simulink model "s_b4a4x64f"  (R2016b)
settings: Solver=VariableStepDiscrete  StartTime=0.0  StopTime=1  RelTol=1e-3
undefined symbols (not defined in the file): fft_stages, n_bits_ants, n_bits_xengs
libraries: xbsIndex_r4 x19869, casper_library_misc x167, casper_library_scopes x10, xbsReplacements_r4 x9, casper_library_delays x8, xps_library x3
(part 12 of 173)

== system s_b4a4x64f/sys3 ==
  note: The time out of the pre_process increments
      | by ONE per freq per fengine.
  31->32 : Subsystem  AncestorBlock=casper_library_bus/bus_convert  mask(bus_convert){n_bits_in=[31 31 31 31 31 31 31 31], bin_pt_in=0, cmplx=off, n_bits_out=32, bin_pt_out=0, quantization=0, overflow=0, latency=0, of=off, misc=off}
      mask prompts: n_bits_in "input bit widths"; bin_pt_in "input binary points"; cmplx "input complex"; n_bits_out "output bit widths"; bin_pt_out "output binary points"; quantization "quantization strategy (Truncate=0, Round  (unbiased: +/- Inf)=1, Round (unbiased: Even Values)=2)"; overflow "overflow strategy (Wrap=0, Saturate=1, Flag as error=2)"; of "overflow indication"; misc "misc support"
      mask help: Convert components of busses
      mask init: same as s_b4a4x64f/sys0/31->32
  Concat1 : xbsIndex_r4/Concat  num_inputs=2  dbl_ovrd=off  block_type=concat
      settings: block_version=10.1.3
  Concat10 : xbsIndex_r4/Concat  num_inputs=2  dbl_ovrd=off  block_type=concat
  Concat11 : xbsIndex_r4/Concat  num_inputs=3  dbl_ovrd=off  block_type=concat
  Concat6 : xbsIndex_r4/Concat  num_inputs=2  dbl_ovrd=off  block_type=concat
  Constant10 : xbsIndex_r4/Constant  const=xeng_id  gui_display_data_type=Fixed-point  arith_type=Unsigned  n_bits=n_bits_xengs_per_fpga  bin_pt=0  preci_type=Single  exp_width=8  frac_width=24  explicit_period=on  period=1  equ=P=C  opselect=C  inp2=PCIN>>17  opr=+  inp1=P  carry=CIN  dbl_ovrd=off  block_type=constant
  Constant11 : xbsIndex_r4/Constant  const=0  gui_display_data_type=Fixed-point  arith_type=Boolean  n_bits=1  bin_pt=0  preci_type=Single  exp_width=8  frac_width=24  explicit_period=on  period=1  equ=P=C  opselect=C  inp2=PCIN>>17  opr=+  inp1=P  carry=CIN  dbl_ovrd=off  block_type=constant
      settings: block_version=11.3
  Constant12 : xbsIndex_r4/Constant  const=0  gui_display_data_type=Fixed-point  arith_type=Boolean  n_bits=1  bin_pt=0  preci_type=Single  exp_width=8  frac_width=24  explicit_period=on  period=1  equ=P=C  opselect=C  inp2=PCIN>>17  opr=+  inp1=P  carry=CIN  dbl_ovrd=off  block_type=constant
      settings: block_version=11.3
  Constant13 : xbsIndex_r4/Constant  const=0  gui_display_data_type=Fixed-point  arith_type=Unsigned  n_bits=n_bits_channels + 1 + x_acc_bits  bin_pt=0  preci_type=Single  exp_width=8  frac_width=24  explicit_period=on  period=1  equ=P=C  opselect=C  inp2=PCIN>>17  opr=+  inp1=P  carry=CIN  dbl_ovrd=off  block_type=constant
  Constant14 : xbsIndex_r4/Constant  const=0  gui_display_data_type=Fixed-point  arith_type=Unsigned  n_bits=16  bin_pt=0  preci_type=Single  exp_width=8  frac_width=24  explicit_period=on  period=1  equ=P=C  opselect=C  inp2=PCIN>>17  opr=+  inp1=P  carry=CIN  dbl_ovrd=off  block_type=constant
  Constant15 : xbsIndex_r4/Constant  const=0  gui_display_data_type=Fixed-point  arith_type=Unsigned  n_bits=16-n_bits_channels  bin_pt=0  preci_type=Single  exp_width=8  frac_width=24  explicit_period=on  period=1  equ=P=C  opselect=C  inp2=PCIN>>17  opr=+  inp1=P  carry=CIN  dbl_ovrd=off  block_type=constant
  Constant5 : xbsIndex_r4/Constant  const=0  gui_display_data_type=Fixed-point  arith_type=Unsigned  n_bits=n_bits_channels + 1 + x_acc_bits  bin_pt=0  preci_type=Single  exp_width=8  frac_width=24  explicit_period=on  period=1  equ=P=C  opselect=C  inp2=PCIN>>17  opr=+  inp1=P  carry=CIN  dbl_ovrd=off  block_type=constant
  Delay{1..4} (4 alike) : xbsIndex_r4/Delay  rst=off  infoeditControl=Selection of Reset will increase slice count due to use of real FFs and instead of SRLs  en=on  latency=1  reg_retiming=on  dbl_ovrd=off  block_type=delay
  Delay10 : Subsystem  AncestorBlock=casper_library_delays/pipeline  mask(pipeline){latency=2}
      mask help:
      | An explicitly laid-out delay line to avoid mapping to SRL16s
      | for use in pipelining to help achieve timing closure.
      mask init:
      | pipeline_init(gcb,'latency',latency);
      settings: AttributesFormatString=Latency = %<latency>
      mask Display:
      | port_label('input', 1, 'd');
      | port_label('output', 1, 'q');
      | disp(['Z^-', num2str(latency)]);
  Delay11 : Subsystem  AncestorBlock=casper_library_delays/pipeline  mask(pipeline){latency=2}
      mask help:
      | An explicitly laid-out delay line to avoid mapping to SRL16s
      | for use in pipelining to help achieve timing closure.
      mask init:
      | pipeline_init(gcb,'latency',latency);
      settings: AttributesFormatString=Latency = %<latency>
      mask Display:
      | port_label('input', 1, 'd');
      | port_label('output', 1, 'q');
      | disp(['Z^-', num2str(latency)]);
  Delay12 : Subsystem  AncestorBlock=casper_library_delays/pipeline  mask(pipeline){latency=2}
      mask help:
      | An explicitly laid-out delay line to avoid mapping to SRL16s
      | for use in pipelining to help achieve timing closure.
      mask init:
      | pipeline_init(gcb,'latency',latency);
      settings: AttributesFormatString=Latency = %<latency>
      mask Display:
      | port_label('input', 1, 'd');
      | port_label('output', 1, 'q');
      | disp(['Z^-', num2str(latency)]);
  Delay13 : Subsystem  AncestorBlock=casper_library_delays/pipeline  mask(pipeline){latency=2}
      mask help:
      | An explicitly laid-out delay line to avoid mapping to SRL16s
      | for use in pipelining to help achieve timing closure.
      mask init:
      | pipeline_init(gcb,'latency',latency);
      settings: AttributesFormatString=Latency = %<latency>
      mask Display:
      | port_label('input', 1, 'd');
      | port_label('output', 1, 'q');
      | disp(['Z^-', num2str(latency)]);
  Delay14 : Subsystem  AncestorBlock=casper_library_delays/pipeline  mask(pipeline){latency=2}
      mask help:
      | An explicitly laid-out delay line to avoid mapping to SRL16s
      | for use in pipelining to help achieve timing closure.
      mask init:
      | pipeline_init(gcb,'latency',latency);
      settings: AttributesFormatString=Latency = %<latency>
      mask Display:
      | port_label('input', 1, 'd');
      | port_label('output', 1, 'q');
      | disp(['Z^-', num2str(latency)]);
  Delay15 : Subsystem  AncestorBlock=casper_library_delays/pipeline  mask(pipeline){latency=2}
      mask help:
      | An explicitly laid-out delay line to avoid mapping to SRL16s
      | for use in pipelining to help achieve timing closure.
      mask init:
      | pipeline_init(gcb,'latency',latency);
      settings: AttributesFormatString=Latency = %<latency>
      mask Display:
      | port_label('input', 1, 'd');
      | port_label('output', 1, 'q');
      | disp(['Z^-', num2str(latency)]);
  Delay16 : Subsystem  AncestorBlock=casper_library_delays/pipeline  mask(pipeline){latency=2}
      mask help:
      | An explicitly laid-out delay line to avoid mapping to SRL16s
      | for use in pipelining to help achieve timing closure.
      mask init:
      | pipeline_init(gcb,'latency',latency);
      settings: AttributesFormatString=Latency = %<latency>
      mask Display:
      | port_label('input', 1, 'd');
      | port_label('output', 1, 'q');
      | disp(['Z^-', num2str(latency)]);
  Delay17 : Subsystem  AncestorBlock=casper_library_delays/pipeline  mask(pipeline){latency=2}
      mask help:
      | An explicitly laid-out delay line to avoid mapping to SRL16s
      | for use in pipelining to help achieve timing closure.
      mask init:
      | pipeline_init(gcb,'latency',latency);
      settings: AttributesFormatString=Latency = %<latency>
      mask Display:
      | port_label('input', 1, 'd');
      | port_label('output', 1, 'q');
      | disp(['Z^-', num2str(latency)]);
  Delay18 : Subsystem  AncestorBlock=casper_library_delays/pipeline  mask(pipeline){latency=2}
      mask help:
      | An explicitly laid-out delay line to avoid mapping to SRL16s
      | for use in pipelining to help achieve timing closure.
      mask init:
      | pipeline_init(gcb,'latency',latency);
      settings: AttributesFormatString=Latency = %<latency>
      mask Display:
      | port_label('input', 1, 'd');
      | port_label('output', 1, 'q');
      | disp(['Z^-', num2str(latency)]);
  Delay19 : Subsystem  AncestorBlock=casper_library_delays/pipeline  mask(pipeline){latency=2}
      mask help:
      | An explicitly laid-out delay line to avoid mapping to SRL16s
      | for use in pipelining to help achieve timing closure.
      mask init:
      | pipeline_init(gcb,'latency',latency);
      settings: AttributesFormatString=Latency = %<latency>
      mask Display:
      | port_label('input', 1, 'd');
      | port_label('output', 1, 'q');
      | disp(['Z^-', num2str(latency)]);
  Delay20 : Subsystem  AncestorBlock=casper_library_delays/pipeline  mask(pipeline){latency=2}
      mask help:
      | An explicitly laid-out delay line to avoid mapping to SRL16s
      | for use in pipelining to help achieve timing closure.
      mask init:
      | pipeline_init(gcb,'latency',latency);
      settings: AttributesFormatString=Latency = %<latency>
      mask Display:
      | port_label('input', 1, 'd');
      | port_label('output', 1, 'q');
      | disp(['Z^-', num2str(latency)]);
  Delay21 : Subsystem  AncestorBlock=casper_library_delays/pipeline  mask(pipeline){latency=2}
      mask help:
      | An explicitly laid-out delay line to avoid mapping to SRL16s
      | for use in pipelining to help achieve timing closure.
      mask init:
      | pipeline_init(gcb,'latency',latency);
      settings: AttributesFormatString=Latency = %<latency>
      mask Display:
      | port_label('input', 1, 'd');
      | port_label('output', 1, 'q');
      | disp(['Z^-', num2str(latency)]);
  Delay22 : Subsystem  AncestorBlock=casper_library_delays/pipeline  mask(pipeline){latency=2}
      mask help:
      | An explicitly laid-out delay line to avoid mapping to SRL16s
      | for use in pipelining to help achieve timing closure.
      mask init:
      | pipeline_init(gcb,'latency',latency);
      settings: AttributesFormatString=Latency = %<latency>
      mask Display:
      | port_label('input', 1, 'd');
      | port_label('output', 1, 'q');
      | disp(['Z^-', num2str(latency)]);
  Delay23 : Subsystem  AncestorBlock=casper_library_delays/pipeline  mask(pipeline){latency=2}
      mask help:
      | An explicitly laid-out delay line to avoid mapping to SRL16s
      | for use in pipelining to help achieve timing closure.
      mask init:
      | pipeline_init(gcb,'latency',latency);
      settings: AttributesFormatString=Latency = %<latency>
      mask Display:
      | port_label('input', 1, 'd');
      | port_label('output', 1, 'q');
      | disp(['Z^-', num2str(latency)]);
  Delay{6..7,32..34,68,71,93} (8 alike) : xbsIndex_r4/Delay  rst=off  infoeditControl=Selection of Reset will increase slice count due to use of real FFs and instead of SRLs  en=off  latency=1  reg_retiming=on  dbl_ovrd=off  block_type=delay
      Delay32 settings: block_version=11.4
      Delay33 settings: block_version=11.4
      Delay34 settings: block_version=11.4
      Delay68 settings: block_version=11.4
      Delay71 settings: block_version=11.4
      Delay93 settings: block_version=11.4
  Delay37 : Subsystem  AncestorBlock=casper_library_delays/pipeline  mask(pipeline){latency=1}
      mask help:
      | An explicitly laid-out delay line to avoid mapping to SRL16s
      | for use in pipelining to help achieve timing closure.
      mask init:
      | pipeline_init(gcb,'latency',latency);
      settings: AttributesFormatString=Latency = %<latency>
      mask Display:
      | port_label('input', 1, 'd');
      | port_label('output', 1, 'q');
      | disp(['Z^-', num2str(latency)]);
  Delay38 : Subsystem  AncestorBlock=casper_library_delays/pipeline  mask(pipeline){latency=1}
      mask help:
      | An explicitly laid-out delay line to avoid mapping to SRL16s
      | for use in pipelining to help achieve timing closure.
      mask init:
      | pipeline_init(gcb,'latency',latency);
      settings: AttributesFormatString=Latency = %<latency>
      mask Display:
      | port_label('input', 1, 'd');
      | port_label('output', 1, 'q');
      | disp(['Z^-', num2str(latency)]);
  Delay{5,81,90..91} (4 alike) : xbsIndex_r4/Delay  rst=off  infoeditControl=Selection of Reset will increase slice count due to use of real FFs and instead of SRLs  en=off  latency=2  reg_retiming=off  dbl_ovrd=off  block_type=delay
      settings: infoedit=Hardware notes: A delay line is a chain, each link of which is an SRL16 or SRL32 followed by a flip-flop.  xl_area=[0, 0, 0, 0, 0, 0, 0]  block_version=9.2.01
  Delay52 : Subsystem  AncestorBlock=casper_library_delays/pipeline  mask(pipeline){latency=1}
      mask help:
      | An explicitly laid-out delay line to avoid mapping to SRL16s
      | for use in pipelining to help achieve timing closure.
      mask init:
      | pipeline_init(gcb,'latency',latency);
      settings: AttributesFormatString=Latency = %<latency>
      mask Display:
      | port_label('input', 1, 'd');
      | port_label('output', 1, 'q');
      | disp(['Z^-', num2str(latency)]);
  Delay69 : Subsystem  AncestorBlock=casper_library_delays/pipeline  mask(pipeline){latency=2}
      mask help:
      | An explicitly laid-out delay line to avoid mapping to SRL16s
      | for use in pipelining to help achieve timing closure.
      mask init:
      | pipeline_init(gcb,'latency',latency);
      settings: AttributesFormatString=Latency = %<latency>
      mask Display:
      | port_label('input', 1, 'd');
      | port_label('output', 1, 'q');
      | disp(['Z^-', num2str(latency)]);
  Delay74 : Subsystem  AncestorBlock=casper_library_delays/pipeline  mask(pipeline){latency=2}
      mask help:
      | An explicitly laid-out delay line to avoid mapping to SRL16s
      | for use in pipelining to help achieve timing closure.
      mask init:
      | pipeline_init(gcb,'latency',latency);
      settings: AttributesFormatString=Latency = %<latency>
      mask Display:
      | port_label('input', 1, 'd');
      | port_label('output', 1, 'q');
      | disp(['Z^-', num2str(latency)]);
  Delay76 : Subsystem  AncestorBlock=casper_library_delays/pipeline  mask(pipeline){latency=2}
      mask help:
      | An explicitly laid-out delay line to avoid mapping to SRL16s
      | for use in pipelining to help achieve timing closure.
      mask init:
      | pipeline_init(gcb,'latency',latency);
      settings: AttributesFormatString=Latency = %<latency>
      mask Display:
      | port_label('input', 1, 'd');
      | port_label('output', 1, 'q');
      | disp(['Z^-', num2str(latency)]);
  Delay77 : Subsystem  AncestorBlock=casper_library_delays/pipeline  mask(pipeline){latency=2}
      mask help:
      | An explicitly laid-out delay line to avoid mapping to SRL16s
      | for use in pipelining to help achieve timing closure.
      mask init:
      | pipeline_init(gcb,'latency',latency);
      settings: AttributesFormatString=Latency = %<latency>
      mask Display:
      | port_label('input', 1, 'd');
      | port_label('output', 1, 'q');
      | disp(['Z^-', num2str(latency)]);
  Delay8 : Subsystem  AncestorBlock=casper_library_delays/pipeline  mask(pipeline){latency=1}
      mask help:
      | An explicitly laid-out delay line to avoid mapping to SRL16s
      | for use in pipelining to help achieve timing closure.
      mask init:
      | pipeline_init(gcb,'latency',latency);
      settings: AttributesFormatString=Latency = %<latency>
      mask Display:
      | port_label('input', 1, 'd');
      | port_label('output', 1, 'q');
      | disp(['Z^-', num2str(latency)]);
  Delay89 : Subsystem  AncestorBlock=casper_library_delays/pipeline  mask(pipeline){latency=2}
      mask help:
      | An explicitly laid-out delay line to avoid mapping to SRL16s
      | for use in pipelining to help achieve timing closure.
      mask init:
      | pipeline_init(gcb,'latency',latency);
      settings: AttributesFormatString=Latency = %<latency>
      mask Display:
      | port_label('input', 1, 'd');
      | port_label('output', 1, 'q');
      | disp(['Z^-', num2str(latency)]);
  Delay9 : Subsystem  AncestorBlock=casper_library_delays/pipeline  mask(pipeline){latency=2}
      mask help:
      | An explicitly laid-out delay line to avoid mapping to SRL16s
      | for use in pipelining to help achieve timing closure.
      mask init:
      | pipeline_init(gcb,'latency',latency);
      settings: AttributesFormatString=Latency = %<latency>
      mask Display:
      | port_label('input', 1, 'd');
      | port_label('output', 1, 'q');
      | disp(['Z^-', num2str(latency)]);
  Inverter : xbsIndex_r4/Inverter  en=off  latency=0  dbl_ovrd=off  block_type=inv
  Inverter2 : xbsIndex_r4/Inverter  en=off  latency=0  dbl_ovrd=off  block_type=inv
  Inverter3 : xbsIndex_r4/Inverter  en=off  latency=0  dbl_ovrd=off  block_type=inv
  Logical : xbsIndex_r4/Logical  logical_function=AND  inputs=2  en=off  latency=0  precision=Full  arith_type=Unsigned  n_bits=16  bin_pt=0  align_bp=on  dbl_ovrd=off  block_type=logical
  Logical1 : xbsIndex_r4/Logical  logical_function=AND  inputs=2  en=off  latency=1  precision=Full  arith_type=Unsigned  n_bits=16  bin_pt=0  align_bp=on  dbl_ovrd=off  block_type=logical
  Mux : xbsIndex_r4/Mux  inputs=2  en=off  latency=1  precision=Full  arith_type=Unsigned  n_bits=16  bin_pt=14  quantization=Truncate  overflow=Wrap  dbl_ovrd=off  block_type=mux
  Register : xbsIndex_r4/Register  init=0  rst=off  en=on  dbl_ovrd=off  block_type=register
  Register2 : xbsIndex_r4/Register  init=0  rst=off  en=on  dbl_ovrd=off  block_type=register
      settings: block_version=11.4
  Register3 : xbsIndex_r4/Register  init=0  rst=off  en=on  dbl_ovrd=off  block_type=register
      settings: block_version=11.4
  Slice1 : xbsIndex_r4/Slice  nbits=timestamp_bits  boolean_output=off  mode=Upper Bit Location + Width  bit1=0  base1=MSB of Input  bit0=timestamp_bits  base0=LSB of Input  dbl_ovrd=off  block_type=slice
  Slice11 : xbsIndex_r4/Slice  nbits=n_bits_xengs - n_bits_xengs_per_fpga  boolean_output=off  mode=Lower Bit Location + Width  bit1=0  base1=MSB of Input  bit0=0  base0=LSB of Input  dbl_ovrd=off  block_type=slice
      settings: block_version=10.1.3
  Slice12 : xbsIndex_r4/Slice  nbits=16  boolean_output=off  mode=Lower Bit Location + Width  bit1=0  base1=MSB of Input  bit0=0  base0=LSB of Input  dbl_ovrd=off  block_type=slice
  Slice15 : xbsIndex_r4/Slice  nbits=1  boolean_output=on  mode=Upper Bit Location + Width  bit1=0  base1=MSB of Input  bit0=0  base0=LSB of Input  dbl_ovrd=off  block_type=slice
  Slice16 : xbsIndex_r4/Slice  nbits=1  boolean_output=on  mode=Lower Bit Location + Width  bit1=0  base1=LSB of Input  bit0=0  base0=LSB of Input  dbl_ovrd=off  block_type=slice
  Slice2 : xbsIndex_r4/Slice  nbits=16  boolean_output=off  mode=Upper Bit Location + Width  bit1=0  base1=MSB of Input  bit0=0  base0=LSB of Input  dbl_ovrd=off  block_type=slice
  Terminator2 : Terminator
  bf : Subsystem  mask{beng_bits=n_bits_xengs, ant_bits=n_bits_ants, polarisation_bits=1, freq_bits=n_bits_channels, stack_bits=x_acc_bits, n_bits_in=8, bin_pt_in=7, bfpga_bits=2, timestamp_bits=timestamp_bits, n_bits_norm=16, bin_pt_norm=9, n_bits_combine=8+16+1+n_bits_ants, n_bits_requant=16, bin_pt_requant=8, bram_latency=5, add_latency=3, mult_latency=5, beam_bits=0, n_bits_out=8, bin_pt_out=7, conv_latency=3, output_enabled=on}
      mask prompts: beng_bits "b-engines (2^?)"; ant_bits "antennas (2^?)"; polarisation_bits "polarisations (2^?)"; freq_bits "frequencies (2^?)"; stack_bits "stacking factor (2^?)"; n_bits_in "data bits in"; bin_pt_in "binary point in"; bfpga_bits "b-engines on FPGA"; timestamp_bits "timestamp size (bits)"; n_bits_norm "calibration factor data bits"; bin_pt_norm "calibration factor binary point"; n_bits_combine "antenna combination output bit width"; n_bits_requant "requantization factor bit width"; bin_pt_requant "requantization factor binary point"; bram_latency "bram latency"; add_latency "add latency"; beam_bits "beams (2^?)"; n_bits_out "data bits out"; bin_pt_out "binary point out"; conv_latency "convert latency"; output_enabled "output enabled by default?"
      mask help:
      | Frequency domain beamformer
      |
      | b-engines: number of b-engines in system (same as x-engines)
      | stacking factor: the number of consecutive time samples in a data block
      | calibration factor: the complex factor multiplied with the incoming data.
      | The complex value is unique to each beam, input and frequency.
      | Requantization factor: real factor multiplied with the output data before
      | quantization. The value is unique to each beam and frequency.
      | beams: the number of beams per polarisation
      | ouput enabled by default: can be useful for simulation
      mask init:
      | set_param([gcb,'/fbf'], ...
      |     'output_enabled', output_enabled);
      mask Help:
      | Accepts the same channelised data as the CASPER FX correlator x-engine core.
      | Polarisations appear in order in different beams. (for polarisation (0,1), 0 in [0,2...], 1 in [1,3...]).
      | TODO: beam steering.
      | TODO: Stokes output.
      | TODO: accumulation.
  bf_pack_out0 : Subsystem  mask(speadify){spead_msw=64, spead_lsw=48, heap_bits=n_bits_channels-n_bits_xengs+x_acc_bits, group_size_bits=n_bits_xengs, n_bits_chans=n_bits_channels-n_bits_xengs, n_bits_acc=x_acc_bits, bit_width_in=1, bit_width_out=5, packet_bits=12, fabric_clock=225, tx_clock=156.25}
      mask prompts: spead_msw "SPEAD flavour (msw)"; spead_lsw "SPEAD flavour (lsw)"; heap_bits "heap size (2^? input words)"; group_size_bits "max SPEAD heap group size (2^?)"; n_bits_chans "channels processed (2^?)"; n_bits_acc "samples from channel (2^?)"; bit_width_in "word size in (2^? bytes)"; bit_width_out "word size out (2^? bytes)"; packet_bits "packet size out (2^? bytes)"; fabric_clock "fabric clock (MHz)"; tx_clock "transmission clock (MHz)"
      mask help:
      | Transforms input data stream to 10Ge ready SPEAD stream.
      | max SPEAD heap group size is the maximum number of SPEAD sources
      | that may be combined when assembling heaps. n_partitions and partition
      | input ports are then used at runtime to configure this.
  bf_pack_out1 : Subsystem  mask(speadify){spead_msw=64, spead_lsw=48, heap_bits=n_bits_channels-n_bits_xengs+x_acc_bits, group_size_bits=n_bits_xengs, n_bits_chans=n_bits_channels-n_bits_xengs, n_bits_acc=x_acc_bits, bit_width_in=1, bit_width_out=5, packet_bits=12, fabric_clock=225, tx_clock=156.25}
      mask prompts: spead_msw "SPEAD flavour (msw)"; spead_lsw "SPEAD flavour (lsw)"; heap_bits "heap size (2^? input words)"; group_size_bits "max SPEAD heap group size (2^?)"; n_bits_chans "channels processed (2^?)"; n_bits_acc "samples from channel (2^?)"; bit_width_in "word size in (2^? bytes)"; bit_width_out "word size out (2^? bytes)"; packet_bits "packet size out (2^? bytes)"; fabric_clock "fabric clock (MHz)"; tx_clock "transmission clock (MHz)"
      mask help:
      | Transforms input data stream to 10Ge ready SPEAD stream.
      | max SPEAD heap group size is the maximum number of SPEAD sources
      | that may be combined when assembling heaps. n_partitions and partition
      | input ports are then used at runtime to configure this.
  pipeline : Subsystem  AncestorBlock=casper_library_delays/pipeline  mask(pipeline){latency=2}
      mask help:
      | An explicitly laid-out delay line to avoid mapping to SRL16s
      | for use in pipelining to help achieve timing closure.
      mask init:
      | pipeline_init(gcb,'latency',latency);
      settings: AttributesFormatString=Latency = %<latency>
      mask Display:
      | port_label('input', 1, 'd');
      | port_label('output', 1, 'q');
      | disp(['Z^-', num2str(latency)]);
  pipeline1 : Subsystem  AncestorBlock=casper_library_delays/pipeline  mask(pipeline){latency=2}
      mask help:
      | An explicitly laid-out delay line to avoid mapping to SRL16s
      | for use in pipelining to help achieve timing closure.
      mask init:
      | pipeline_init(gcb,'latency',latency);
      settings: AttributesFormatString=Latency = %<latency>
      mask Display:
      | port_label('input', 1, 'd');
      | port_label('output', 1, 'q');
      | disp(['Z^-', num2str(latency)]);
  pipeline10 : Subsystem  AncestorBlock=casper_library_delays/pipeline  mask(pipeline){latency=2}
      mask help:
      | An explicitly laid-out delay line to avoid mapping to SRL16s
      | for use in pipelining to help achieve timing closure.
      mask init:
      | pipeline_init(gcb,'latency',latency);
      settings: AttributesFormatString=Latency = %<latency>
      mask Display:
      | port_label('input', 1, 'd');
      | port_label('output', 1, 'q');
      | disp(['Z^-', num2str(latency)]);
  pipeline11 : Subsystem  AncestorBlock=casper_library_delays/pipeline  mask(pipeline){latency=2}
      mask help:
      | An explicitly laid-out delay line to avoid mapping to SRL16s
      | for use in pipelining to help achieve timing closure.
      mask init:
      | pipeline_init(gcb,'latency',latency);
      settings: AttributesFormatString=Latency = %<latency>
      mask Display:
      | port_label('input', 1, 'd');
      | port_label('output', 1, 'q');
      | disp(['Z^-', num2str(latency)]);
  pipeline12 : Subsystem  AncestorBlock=casper_library_delays/pipeline  mask(pipeline){latency=2}
      mask help:
      | An explicitly laid-out delay line to avoid mapping to SRL16s
      | for use in pipelining to help achieve timing closure.
      mask init:
      | pipeline_init(gcb,'latency',latency);
      settings: AttributesFormatString=Latency = %<latency>
      mask Display:
      | port_label('input', 1, 'd');
      | port_label('output', 1, 'q');
      | disp(['Z^-', num2str(latency)]);
  pipeline13 : Subsystem  AncestorBlock=casper_library_delays/pipeline  mask(pipeline){latency=2}
      mask help:
      | An explicitly laid-out delay line to avoid mapping to SRL16s
      | for use in pipelining to help achieve timing closure.
      mask init:
      | pipeline_init(gcb,'latency',latency);
      settings: AttributesFormatString=Latency = %<latency>
      mask Display:
      | port_label('input', 1, 'd');
      | port_label('output', 1, 'q');
      | disp(['Z^-', num2str(latency)]);
  pipeline14 : Subsystem  AncestorBlock=casper_library_delays/pipeline  mask(pipeline){latency=2}
      mask help:
      | An explicitly laid-out delay line to avoid mapping to SRL16s
      | for use in pipelining to help achieve timing closure.
      mask init:
      | pipeline_init(gcb,'latency',latency);
      settings: AttributesFormatString=Latency = %<latency>
      mask Display:
      | port_label('input', 1, 'd');
      | port_label('output', 1, 'q');
      | disp(['Z^-', num2str(latency)]);
  pipeline2 : Subsystem  AncestorBlock=casper_library_delays/pipeline  mask(pipeline){latency=2}
      mask help:
      | An explicitly laid-out delay line to avoid mapping to SRL16s
      | for use in pipelining to help achieve timing closure.
      mask init:
      | pipeline_init(gcb,'latency',latency);
      settings: AttributesFormatString=Latency = %<latency>
      mask Display:
      | port_label('input', 1, 'd');
      | port_label('output', 1, 'q');
      | disp(['Z^-', num2str(latency)]);
  pipeline3 : Subsystem  AncestorBlock=casper_library_delays/pipeline  mask(pipeline){latency=2}
      mask help:
      | An explicitly laid-out delay line to avoid mapping to SRL16s
      | for use in pipelining to help achieve timing closure.
      mask init:
      | pipeline_init(gcb,'latency',latency);
      settings: AttributesFormatString=Latency = %<latency>
      mask Display:
      | port_label('input', 1, 'd');
      | port_label('output', 1, 'q');
      | disp(['Z^-', num2str(latency)]);
  pipeline4 : Subsystem  AncestorBlock=casper_library_delays/pipeline  mask(pipeline){latency=2}
      mask help:
      | An explicitly laid-out delay line to avoid mapping to SRL16s
      | for use in pipelining to help achieve timing closure.
      mask init:
      | pipeline_init(gcb,'latency',latency);
      settings: AttributesFormatString=Latency = %<latency>
      mask Display:
      | port_label('input', 1, 'd');
      | port_label('output', 1, 'q');
      | disp(['Z^-', num2str(latency)]);
  pipeline5 : Subsystem  AncestorBlock=casper_library_delays/pipeline  mask(pipeline){latency=2}
      mask help:
      | An explicitly laid-out delay line to avoid mapping to SRL16s
      | for use in pipelining to help achieve timing closure.
      mask init:
      | pipeline_init(gcb,'latency',latency);
      settings: AttributesFormatString=Latency = %<latency>
      mask Display:
      | port_label('input', 1, 'd');
      | port_label('output', 1, 'q');
      | disp(['Z^-', num2str(latency)]);
  pipeline6 : Subsystem  AncestorBlock=casper_library_delays/pipeline  mask(pipeline){latency=2}
      mask help:
      | An explicitly laid-out delay line to avoid mapping to SRL16s
      | for use in pipelining to help achieve timing closure.
      mask init:
      | pipeline_init(gcb,'latency',latency);
      settings: AttributesFormatString=Latency = %<latency>
      mask Display:
      | port_label('input', 1, 'd');
      | port_label('output', 1, 'q');
      | disp(['Z^-', num2str(latency)]);
  pipeline7 : Subsystem  AncestorBlock=casper_library_delays/pipeline  mask(pipeline){latency=2}
      mask help:
      | An explicitly laid-out delay line to avoid mapping to SRL16s
      | for use in pipelining to help achieve timing closure.
      mask init:
      | pipeline_init(gcb,'latency',latency);
      settings: AttributesFormatString=Latency = %<latency>
      mask Display:
      | port_label('input', 1, 'd');
      | port_label('output', 1, 'q');
      | disp(['Z^-', num2str(latency)]);
  pipeline8 : Subsystem  AncestorBlock=casper_library_delays/pipeline  mask(pipeline){latency=2}
      mask help:
      | An explicitly laid-out delay line to avoid mapping to SRL16s
      | for use in pipelining to help achieve timing closure.
      mask init:
      | pipeline_init(gcb,'latency',latency);
      settings: AttributesFormatString=Latency = %<latency>
      mask Display:
      | port_label('input', 1, 'd');
      | port_label('output', 1, 'q');
      | disp(['Z^-', num2str(latency)]);
  pipeline9 : Subsystem  AncestorBlock=casper_library_delays/pipeline  mask(pipeline){latency=2}
      mask help:
      | An explicitly laid-out delay line to avoid mapping to SRL16s
      | for use in pipelining to help achieve timing closure.
      mask init:
      | pipeline_init(gcb,'latency',latency);
      settings: AttributesFormatString=Latency = %<latency>
      mask Display:
      | port_label('input', 1, 'd');
      | port_label('output', 1, 'q');
      | disp(['Z^-', num2str(latency)]);
  pkt_reord : Subsystem  mask{ant_bits=n_bits_ants, xeng_bits=n_bits_xengs, chan_bits=n_bits_channels, x_int_bits=x_acc_bits, window_bits=2, min_sync_bits=x_acc_bits+(n_bits_channels-n_bits_xengs)+3, n_bits_timestamp=timestamp_bits, n_bits_data=32, n_bits_input_words=3, n_bits_output_words=0}
      mask prompts: ant_bits "Maximum Number of Antennas (2^?):"; xeng_bits "Number of Xengines in the system (2^?)"; chan_bits "Number of frequency channels in the system (2^?)"; x_int_bits "X Engine Integration Length (2^?):"; window_bits "Number of Windows to Buffer (2^?):"; min_sync_bits "Minimum sync period (2^n)"; n_bits_timestamp "Timestamp bit width"; n_bits_data "Input data word width"; n_bits_input_words "Input data words (2^?)"; n_bits_output_words "Output data words (2^?)"
      mask init: same as s_b4a4x64f/sys0/pkt_reord
      settings: AttributesFormatString=|
      | Sync period: 2^17
      | Payload Len: 64
  pre_process : Subsystem  mask{share_bits=2, xeng_bits=n_bits_xengs, freq_bits=n_bits_channels, acc_bits=x_acc_bits, time_bits=3, ant_bits=n_bits_ants}
      mask prompts: share_bits "Number of X-engines on this link (2^N)?"; xeng_bits "Number of X-engines in system (2^N)?"; freq_bits "Number of frequency channels in system (2^N)?"; acc_bits "xengine accumulation length (2^?)"; time_bits "samples per timestamp increment (2^?)"; ant_bits "max number of antennas in system (2^?)"
  vacc : Subsystem  Tag=casper:vacc  mask{ants_bits=n_bits_ants, freq_bits=fft_stages-1, xeng_bits=n_bits_xengs, acc_bits=x_acc_bits, tick_bits=0, mezz=1, n_inputs=3, n_bits=31, n_bits_flags=ones(1,19)}
      mask prompts: ants_bits "Number of antennas (2^n)"; freq_bits "Number of frequency channels (2^n)"; xeng_bits "Number of X engines (2^n)"; acc_bits "Pre-accumulation in xengine (2^?)"; tick_bits "Timestamp samples per tick (2^?)"; mezz "HMC Mezz site"; n_inputs "Simultaneous inputs (2^?)"; n_bits "Data width (bits)"; n_bits_flags "Flag bit widths"
      mask help: Hardcoded for X engines with a demux of 8!
      mask init: same as s_b4a4x64f/sys0/vacc
      settings: AttributesFormatString=Vector Length: 640
      mask TypeOptions mezz: 0 | 1 | 2 | 3
  vacc_tvg : Subsystem  AncestorBlock=casper_library/Accumulators/vacc_tvg  mask{len=(2^n_bits_ants*(2^n_bits_ants+1))/2*8*2^(n_bits_channels-n_bits_xengs), n_bits=32, n_inputs=8}
      mask prompts: len "Number of Vectors"; n_bits "Data bits"; n_inputs "Simultaneous inputs"
      mask init:
      | fmtstr = sprintf('Vector Length: %d', len/n_inputs);
      | set_param(gcb, 'AttributesFormatString', fmtstr);
      settings: AttributesFormatString=Vector Length: 640
  x_cast : Subsystem  mask{n_bits_in=32, n_bits_out=31, fix_pnt_pos=0, demux_factor=1}
      mask prompts: n_bits_in "Number of bits (input)"; n_bits_out "Number of bits (output)"; fix_pnt_pos "Fixed point position"; demux_factor "Demux Factor"
      mask init: same as s_b4a4x64f/sys0/x_cast
      settings: AttributesFormatString=32 -> 31, demux 1.
  xeng : Subsystem  Tag=casper:xeng  AncestorBlock=casper_library_correlator/xeng  mask(xeng){n_ants=2^n_bits_ants, n_bits=8, acc_len=2^x_acc_bits, demux_factor=1, add_latency=3, mult_latency=4, bram_latency=7, use_ded_mult=1, use_bram_delay=1}
      mask prompts: n_ants "Number of antennas"; n_bits "Bit-width of samples in"; acc_len "Accumulation length"; add_latency "Adder latency"; mult_latency "Multiplier latency"; bram_latency "BRAM latency"; use_ded_mult "Implementation: Multiplier type (0=slices 1=embedded 2=bram)"; use_bram_delay "Implementation: Delay type (0=SLR, 1=BRAM)"
      mask help: CASPER X engine with added internal valid data masking functionality, descramble and integral demux. Based on Aaron Parsons' and Lynn Urry's original X engine design.
      mask init: same as s_b4a4x64f/sys0/xeng
      settings: AttributesFormatString=n_ant=4, bits=8, mult_typ=1, bram_typ=1
      mask TypeOptions demux_factor: 1 | 2 | 4 | 8
  xeng_pack_out : Subsystem  mask(pkt_pack_mask){vector_len=(2^n_bits_ants*(2^n_bits_ants+1))/2*8*2^(n_bits_channels-n_bits_xengs)/8, n_bits_chans=n_bits_channels-n_bits_xengs, n_bits_word_size=5, heap_len=(2^n_bits_ants*(2^n_bits_ants+1))/2*8*(2^(n_bits_channels-n_bits_xengs))*4, fifo_latency=3, spead_msw=64, spead_lsw=48, spead_item=6144, pkt_bits=11-5, n_bits_max_gap=20, n_bits_timestamp_padding=((n_bits_channels + 1 + x_acc_bits)-3)+3}
      mask prompts: vector_len "vector length (words)"; n_bits_chans "frequency channels (2^?)"; n_bits_word_size "word size (2^? bytes)"; heap_len "System heap size (bytes)"; fifo_latency "Fifo Latency"; spead_msw "SPEAD flavour (MSw)"; spead_lsw "SPEAD flavour (LSw)"; spead_item "SPEAD item number"; pkt_bits "desired payload length (2^?) 256-bit words"; n_bits_max_gap "max gap between packets (2^? clock cycles)"; n_bits_timestamp_padding "Timestamp padding"
      mask help:
      | This block generates packets from a datastream.
      |
      | Packets are created with a fixed header followed by a user-specified number of 64-bit options.
      |
      | Requires a 64-bit data stream.
      |
      | System head size: number of baselines * number of stokes values * number of words per stokes value * number of frequencies * number of bytes per word
      |
      | See the documentation for further details.
      mask init:
      | vector_bits = ceil(log2(vector_len));
      | pkt_len=2^(pkt_bits);
      | fmtstr = sprintf('Vector Length: %d', vector_len);
      | set_param(gcb, 'AttributesFormatString', fmtstr);
      settings: AttributesFormatString=Vector Length: 640
  xeng_tvg : Subsystem  AncestorBlock=casper_library/Correlator/xeng_tvg  mask{n_bits=8, ant_bits=n_bits_ants, x_int_bits=x_acc_bits, sync_period=8+(n_bits_channels-n_bits_xengs)+4, mcnt_period=8+(n_bits_channels-n_bits_xengs), mcnt_step=(n_bits_channels+1-3)+8, n_bits_mcnt=timestamp_bits}
      mask prompts: n_bits "Data bits"; ant_bits "Number of Antennas (2^?):"; x_int_bits "X Integration Length (2^?):"; sync_period "Sync Pulse Period (2^?):"; mcnt_period "Mcnt period (2^?)"; mcnt_step "Mcnt step (2^?)"; n_bits_mcnt "Mcnt bit width (2^?)"
  tag scope: bf0s_d3=global, bf0s_en3=global, bf0s_eof3=global, bf0s_pkt_ready3=global, bf1s_d3=global, bf1s_en3=global, bf1s_eof3=global, bf1s_pkt_ready3=global, bfout_d3=global, bfout_den3=global, bfout_sync3=global, bfout_time3=global, bfout_valbw3=global, id3=global, pack_err3=global, pack_fetch3=global, pack_ready3=global, pack_txd3=global, pack_txeof3=global, pack_txvld3=global, pre_data_3=global, pre_feng_id_3=global, pre_freq_3=global, pre_pkt_idx_3=global, pre_timestamp_3=global, pre_valid_3=global, reord_data3=global, reord_freq3=global, reord_pktdisc3=global, reord_recv3=global, reord_recverr3=global, reord_sync3=global, reord_time3=global, reord_timeouterr3=global, reord_valid3=global, vacc_data3=global, vacc_err3=global, vacc_pktrdy3=global, vacc_rbdone3=global, vacc_time3=global, vacc_valid3=global, vaccin_arm3=global, vaccin_data3=global, vaccin_rst3=global, vaccin_sync3=global, vaccin_time3=global, vaccin_valid3=global
  wires:
  [vacc_time3] -> Concat1/1
  Concat1/1 -> xeng_pack_out/5(timestamp)
  Constant5/1 -> Concat1/2
  Slice1/1 -> vacc/3(start_time)
  Constant15/1 -> Concat11/1
  [reord_freq3] -> Concat11/2
  Constant14/1 -> Concat11/3
  Concat10/1 -> [bfout_time3]
  pipeline12/1(q) -> Concat10/1
  Constant13/1 -> Concat10/2
  Mux/1 -> bf/1(di)
  Delay52/1(q) -> Mux/1
  [bf_tvgsel] -> Delay52/1(d)
  Concat11/1 -> Mux/3
  [reord_data3] -> Mux/2
  Delay93/1 -> [bf0s_en3]
  pipeline14/1(q) -> [bfout_valbw3]
  pipeline13/1(q) -> Terminator2/1
  pipeline11/1(q) -> [bfout_den3]
  pipeline9/1(q) -> [bfout_d3]
  pipeline8/1(q) -> [bfout_sync3]
  [bfout_time3] -> bf_pack_out1/5(timei), bf_pack_out0/5(timei)
  [bfout_den3] -> Slice15/1, Slice16/1
  [bfout_d3] -> Slice2/1, Slice12/1
  [bfout_sync3] -> bf_pack_out1/2(synci), bf_pack_out0/2(synci)
  Delay37/1(q) -> bf/2(deni)
  [reord_time3] -> Delay38/1(d)
  Delay38/1(q) -> bf/4(timei)
  Slice12/1 -> bf_pack_out1/3(di)
  bf_pack_out1/4(pkt_ready) -> Delay33/1
  bf_pack_out1/3(eofo) -> Delay32/1
  bf_pack_out1/2(eno) -> Register3/2, Delay34/1
  bf_pack_out1/1(do) -> Register3/1
  [bf1_tx_pkt3] -> bf_pack_out1/6(start)
  Delay33/1 -> [bf1s_pkt_ready3]
  Register3/1 -> [bf1s_d3]
  bf_pack_out0/4(pkt_ready) -> Delay71/1
  bf_pack_out0/3(eofo) -> Delay68/1
  bf_pack_out0/2(eno) -> Register2/2, Delay93/1
  bf_pack_out0/1(do) -> Register2/1
  Slice15/1 -> bf_pack_out0/4(eni)
  Delay71/1 -> [bf0s_pkt_ready3]
  Delay68/1 -> [bf0s_eof3]
  Register2/1 -> [bf0s_d3]
  [reord_valid3] -> Delay37/1(d)
  Slice16/1 -> bf_pack_out1/4(eni)
  Slice2/1 -> bf_pack_out0/3(di)
  Constant12/1 -> bf/5(misci)
  Constant11/1 -> bf/3(badi)
  [board_id] -> Slice11/1
  Concat6/1 -> [id3]
  Slice11/1 -> Concat6/1
  Constant10/1 -> Concat6/2
  [gap_size3] -> xeng_pack_out/8(gap_size)
  vacc/6(pkt_rdy) -> pipeline4/1(d)
  vacc/2(valid_out) -> pipeline1/1(d)
  vacc/1(data_out) -> pipeline/1(d)
  pipeline10/1(q) -> vacc/9(timestamp_in)
  pipeline7/1(q) -> vacc/8(we)
  pipeline6/1(q) -> vacc/7(data_in)
  pipeline5/1(q) -> vacc/6(sync_in)
  vacc_tvg/4(misco) -> pipeline10/1(d), [vaccin_time3]
  xeng_pack_out/5(fetch) -> [pack_fetch3]
  [go3] -> xeng_pack_out/7(go)
  [id3] -> xeng_pack_out/6(xeng_id)
  [vacc_pktrdy3] -> xeng_pack_out/3(pkt_rdy)
  xeng_pack_out/6(pkt_ready) -> [pack_ready3]
  Delay77/1(q) -> Logical/2
  Logical/1 -> [pack_txvld3]
  xeng_pack_out/2(valid_out) -> Delay77/1(d)
  Register/1 -> Logical/1
  [gbe_txen] -> Register/1
  Delay74/1(q) -> [pack_txd3]
  Delay69/1(q) -> Register/2, [pack_txeof3]
  Delay76/1(q) -> [pack_err3]
  xeng_pack_out/4(err) -> Delay76/1(d)
  xeng_pack_out/1(data_out) -> Delay74/1(d)
  [vacc_rbdone3] -> xeng_pack_out/4(rb_done)
  [vacc_valid3] -> xeng_pack_out/2(valid_in)
  [vacc_data3] -> 31->32/1(din)
  xeng_pack_out/3(eof) -> Delay69/1(d)
  vacc_tvg/1(sync_out) -> pipeline5/1(d), [vaccin_sync3]
  vacc_tvg/3(valid_out) -> pipeline7/1(d), [vaccin_valid3]
  [acc_len] -> vacc/5(acc_len)
  [vacc_ld_arm] -> vacc/2(arm), [vaccin_arm3]
  [vacc_ld_time] -> Slice1/1
  [cnt_rst] -> vacc/1(cnt_rst), [vaccin_rst3]
  [vacc_ld_immediate] -> vacc/4(immediate)
  pipeline3/1(q) -> [vacc_time3]
  pipeline2/1(q) -> [vacc_rbdone3]
  pipeline1/1(q) -> [vacc_valid3]
  pipeline/1(q) -> [vacc_data3]
  Delay8/1(q) -> [reord_recverr3]
  Delay21/1(q) -> [reord_recv3]
  Logical1/1 -> Delay8/1(d)
  Inverter/1 -> Logical1/1
  pkt_reord/6(recvd) -> Delay21/1(d), Inverter/1
  Delay7/1 -> pkt_reord/3(pkt_idx)
  Delay6/1 -> pkt_reord/2(valid_in)
  [pre_freq_3] -> Delay4/1
  [pre_feng_id_3] -> Delay3/1
  [pre_data_3] -> Delay1/1
  [pre_timestamp_3] -> Delay2/1
  Delay2/1 -> pkt_reord/4(time)
  Delay4/1 -> pkt_reord/6(freq)
  Delay3/1 -> pkt_reord/5(ant)
  Delay1/1 -> pkt_reord/1(din)
  pkt_reord/8(mcnt_timeout) -> Delay89/1(d)
  Delay89/1(q) -> [reord_timeouterr3]
  Delay22/1(q) -> [reord_pktdisc3]
  Delay23/1(q) -> [reord_freq3]
  Delay18/1(q) -> [reord_time3]
  Delay16/1(q) -> [reord_valid3]
  Delay15/1(q) -> [reord_data3]
  Delay20/1(q) -> [reord_sync3]
  pkt_reord/7(packet_discarded) -> Delay22/1(d)
  pkt_reord/5(freq_out) -> Delay23/1(d)
  pkt_reord/4(time_out) -> Delay18/1(d)
  pkt_reord/3(valid_out) -> Delay16/1(d), Logical1/2
  pkt_reord/2(data_out) -> Delay15/1(d)
  pkt_reord/1(sync_out) -> Delay20/1(d)
  [id3] -> pkt_reord/7(xeng_id)
  [pre_pkt_idx_3] -> Delay7/1
  [pre_valid_3] -> Delay6/1, Delay2/2, Delay3/2, Delay4/2, Delay1/2
  vacc_tvg/2(data_out) -> x_cast/1(in)
  [pack_fetch3] -> vacc/10(re)
  vacc/3(rb_done) -> pipeline2/1(d)
  vacc/4(timestamp_out) -> pipeline3/1(d)
  vacc/5(error_out) -> [vacc_err3]
  pre_process/1(data_out) -> [pre_data_3]
  pre_process/2(valid) -> [pre_valid_3]
  pre_process/3(eof_out) -> [pre_pkt_idx_3]
  pre_process/4(timestamp) -> [pre_timestamp_3]
  pre_process/5(feng_id) -> [pre_feng_id_3]
  pre_process/6(freq_out) -> [pre_freq_3]
  [id3] -> bf_pack_out0/7(id)
  [bf0_tx_pkt3] -> bf_pack_out0/6(start)
  [id3] -> bf_pack_out1/7(id)
  x_cast/1(out) -> pipeline6/1(d), [vaccin_data3]
  31->32/1(dout) -> xeng_pack_out/1(data_in)
  pipeline4/1(q) -> [vacc_pktrdy3]
  bf/1(synco) -> pipeline8/1(d)
  bf/2(do) -> pipeline9/1(d)
  bf/3(deno) -> pipeline11/1(d)
  bf/4(timeo) -> pipeline12/1(d)
  bf/5(misco) -> pipeline13/1(d)
  bf/6(value_out_bw) -> pipeline14/1(d)
  xeng/3(acc) -> Delay90/1
  xeng/4(mcnt_out) -> Delay91/1
  xeng_tvg/1(sync_out) -> xeng/1(sync_in)
  xeng_tvg/2(data_out) -> xeng/2(ant)
  xeng_tvg/3(valid_out) -> xeng/3(window_valid)
  xeng_tvg/4(mcnto) -> xeng/4(mcnt_in)
  xeng/2(valid) -> Delay5/1
  xeng/1(sync_out) -> Delay81/1
  Delay91/1 -> vacc_tvg/4(misci)
  Delay90/1 -> vacc_tvg/3(data_in)
  Delay5/1 -> vacc_tvg/2(valid_in)
  Delay81/1 -> vacc_tvg/1(sync_in)
  [reord_valid3] -> xeng_tvg/3(valid_in)
  [reord_time3] -> xeng_tvg/4(mcnti)
  [reord_data3] -> xeng_tvg/2(data_in)
  [reord_sync3] -> xeng_tvg/1(sync)
  Delay32/1 -> [bf1s_eof3]
  Delay34/1 -> [bf1s_en3]
  [bf0_txen] -> Inverter2/1
  [bf1_txen] -> Inverter3/1
  Inverter3/1 -> bf_pack_out1/1(rst)
  Inverter2/1 -> bf_pack_out0/1(rst)
  Delay14/1(q) -> pre_process/4(spead_time48)
  Delay19/1(q) -> pre_process/8(freq_in)
  Delay17/1(q) -> pre_process/5(spead_fengid)
  Delay12/1(q) -> pre_process/2(valid_in)
  Delay10/1(q) -> pre_process/7(this_xeng_id)
  Delay9/1(q) -> pre_process/6(dest_xeng)
  Delay11/1(q) -> pre_process/1(data_in)
  Delay13/1(q) -> pre_process/3(eof_in)
  [hmc_reord_data] -> Delay11/1(d)
  [hmc_reord_valid] -> Delay12/1(d)
  [hmc_reord_pkt_idx] -> Delay13/1(d)
  [hmc_reord_timestamp] -> Delay14/1(d)
  [hmc_reord_fengid] -> Delay17/1(d)
  [id3] -> Delay10/1(d)
  [hmc_reord_freq] -> Delay19/1(d)
  [hmc_reord_xeng] -> Delay9/1(d)
